simulink model "control_tsc_planta"  (R2024a)
settings: Solver=ode15s  StartTime=0.0  StopTime=tm_final  MaxStep=tm_h  RelTol=1e-9  AbsTol=1e-11
model workspace (MAT data in the model file):
  tm_C1 = 1.87501784269e-05
  tm_C2 = 3.75003568539e-05
  tm_Cp = 2.89288467158e-06
  tm_L1 = 0.26018031666
  tm_L2 = 0.13009015833
  tm_PNominal_W = 1000
  tm_R1 = 1.15690788571
  tm_R2 = 0.578453942857
  tm_Rb1 = 84640
  tm_Rb2 = 42320
  tm_Rp = 2.20064
  tm_Urms = 230
  tm_a1 = 1
  tm_a2 = 0.03
  tm_a3 = 0.03
  tm_carga = [0 0.0001 0.0002 0.0003 0.0004 0.0005 0.0006 0.0007 0.0008 0.0009 0.001 0.0011 ... (16020 elements, 8010x2)]
  tm_final = 0.8
  tm_h = 2.5e-05
  tm_lambda = 229.793279031
  tm_modes = [0 0.0351508783586 0.0351508783586 0.248585882825 0.248585882825 0.255150878358 0.255150878358 0.3300515321 0.3300515321 0.450321519106 0.450321519106 0.530051552275 ... (60 elements, 20x3)]
  tm_omega = 314.159265359
  tm_outputtimes = [0 0.0001 0.0002 0.0003 0.0004 0.0005 0.0006 0.0007 0.0008 0.0009 0.001 0.0011 ... (8014 elements, 8014x1)]
  tm_vC10 = 0
  tm_vC20 = 0
  tm_vCp0 = 344.473571203
(part 2 of 2)

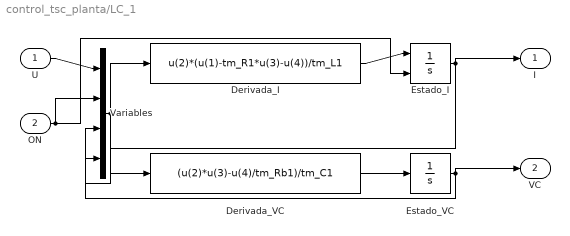
== system control_tsc_planta/LC_1 ==
  U : Inport
  ON : Inport  Port=2
  Derivada_I : Fcn  Expr=u(2)*(u(1)-tm_R1*u(3)-u(4))/tm_L1
  Derivada_VC : Fcn  Expr=(u(2)*u(3)-u(4)/tm_Rb1)/tm_C1
  Estado_I : Integrator  ExternalReset=falling
  Estado_VC : Integrator  InitialCondition=tm_vC10
  Variables : Mux
  I : Outport
  VC : Outport  Port=2
  wires:
  U/1 -> Variables/1
  ON/1 -> Variables/2, Estado_I/2
  Estado_I/1 -> Variables/3, I/1
  Estado_VC/1 -> Variables/4, VC/1
  Variables/1 -> Derivada_I/1, Derivada_VC/1
  Derivada_I/1 -> Estado_I/1
  Derivada_VC/1 -> Estado_VC/1

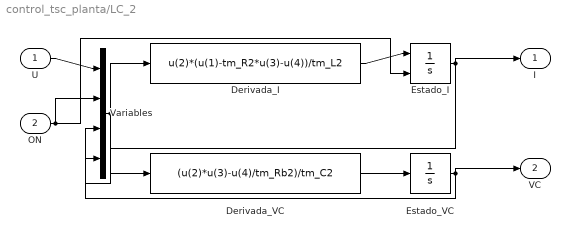
== system control_tsc_planta/LC_2 ==
  U : Inport
  ON : Inport  Port=2
  Derivada_I : Fcn  Expr=u(2)*(u(1)-tm_R2*u(3)-u(4))/tm_L2
  Derivada_VC : Fcn  Expr=(u(2)*u(3)-u(4)/tm_Rb2)/tm_C2
  Estado_I : Integrator  ExternalReset=falling
  Estado_VC : Integrator  InitialCondition=tm_vC20
  Variables : Mux
  I : Outport
  VC : Outport  Port=2
  wires:
  U/1 -> Variables/1
  ON/1 -> Variables/2, Estado_I/2
  Estado_I/1 -> Variables/3, I/1
  Estado_VC/1 -> Variables/4, VC/1
  Variables/1 -> Derivada_I/1, Derivada_VC/1
  Derivada_I/1 -> Estado_I/1
  Derivada_VC/1 -> Estado_VC/1
